simulink model "nonlinear_MPC"  (R2026a)
settings: Solver=ode23s  StopTime=1369
undefined symbols (not defined in the file): acp, bcp, c, ccp, dcp, f, ka, kc, Pamb, R, Ra, T, va, vc
libraries: autolibrcnetworksystem x1, mpclib x1
settings Model: Creator=siddh  LastModifiedBy=siddh

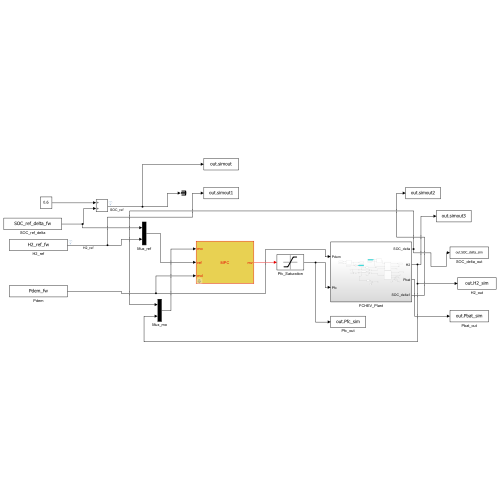
[thumbnail: Simulink's stored preview of the top-level diagram]
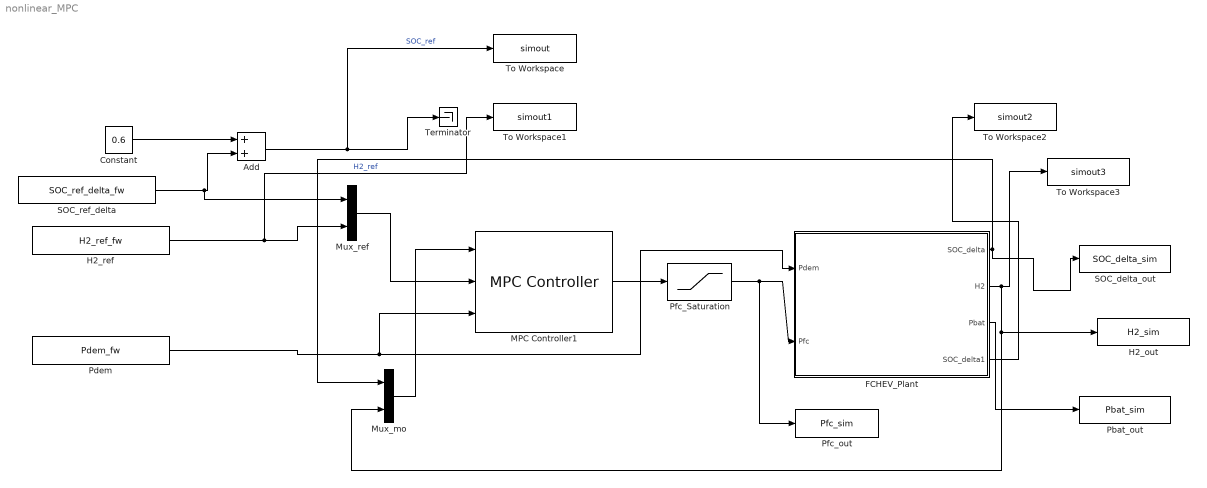
== system nonlinear_MPC ==
  Add : Sum
  Constant : Constant  Value=0.6
  FCHEV_Plant : Subsystem
  H2_out : ToWorkspace  VariableName=H2_sim  SaveFormat=Timeseries  SampleTime=-1
  H2_ref : FromWorkspace  VariableName=H2_ref_fw  SampleTime=-1  OutputAfterFinalValue=Holding final value
  MPC Controller1 : mpclib/MPC Controller  SCDEnableBlockLinearizationSpecification=on  mpcobj=mpcobj  is_multiple=0  enable_value=0  return_u0=off  updateMPCinCallerWorkspace=on  md_inport=on  mv_inport=off  uref_inport=off  return_cost=off  return_mvseq=off  return_qpstatus=off  return_xseq=off  return_state=off  return_ovseq=off  state_inport=off  umin_inport=off  umax_inport=off  ymin_inport=off  ymax_inport=off  cc_inport=off  ywt_inport=off  uwt_inport=off  duwt_inport=off  rhoeps_inport=off  pm_inport=off  MaximumP=10  HorizonChoice=FixedHorizon  n_ts=1  n_p=30  n_mv=1  n_md=1  n_ud=0  n_mo=2  n_uo=0  BlockDataType=double  SampleTimeInherited=off  switch_inport=off
  Mux_mo : Mux  Inputs=2
  Mux_ref : Mux  Inputs=2
  Pbat_out : ToWorkspace  VariableName=Pbat_sim  SaveFormat=Timeseries  SampleTime=-1
  Pdem : FromWorkspace  VariableName=Pdem_fw  SampleTime=-1  OutputAfterFinalValue=Holding final value
  Pfc_Saturation : Saturate  UpperLimit=106000  LowerLimit=0
  Pfc_out : ToWorkspace  VariableName=Pfc_sim  SaveFormat=Timeseries  SampleTime=-1
  SOC_delta_out : ToWorkspace  VariableName=SOC_delta_sim  SaveFormat=Timeseries  SampleTime=-1
  SOC_ref_delta : FromWorkspace  VariableName=SOC_ref_delta_fw  SampleTime=-1  OutputAfterFinalValue=Holding final value
  Terminator : Terminator
  To Workspace : ToWorkspace  VariableName=simout  SaveFormat=Timeseries  SampleTime=-1
  To Workspace1 : ToWorkspace  VariableName=simout1  SaveFormat=Timeseries  SampleTime=-1
  To Workspace2 : ToWorkspace  VariableName=simout2  SaveFormat=Timeseries  SampleTime=-1
  To Workspace3 : ToWorkspace  VariableName=simout3  SaveFormat=Timeseries  SampleTime=-1
  wires:
  H2_ref/1 -> To Workspace1/1, Mux_ref/2  "H2_ref"
  Mux_ref/1 -> MPC Controller1/2
  Pdem/1 -> MPC Controller1/3, FCHEV_Plant/1(Pdem)
  MPC Controller1/1 -> Pfc_Saturation/1
  Pfc_Saturation/1 -> FCHEV_Plant/2(Pfc), Pfc_out/1
  FCHEV_Plant/1(SOC_delta) -> SOC_delta_out/1, Mux_mo/1
  FCHEV_Plant/2(H2) -> To Workspace3/1, Mux_mo/2, H2_out/1
  Mux_mo/1 -> MPC Controller1/1
  FCHEV_Plant/3(Pbat) -> Pbat_out/1
  SOC_ref_delta/1 -> Mux_ref/1, Add/2
  Constant/1 -> Add/1
  Add/1 -> To Workspace/1, Terminator/1  "SOC_ref"
  FCHEV_Plant/4(SOC_delta1) -> To Workspace2/1

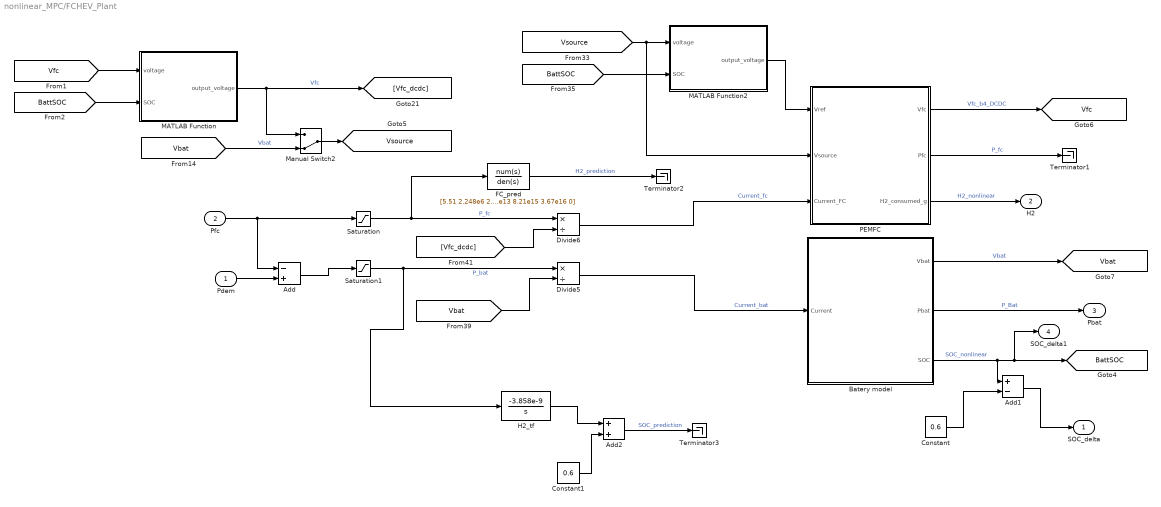
== system nonlinear_MPC/FCHEV_Plant ==
  Pdem : Inport
  Pfc : Inport  Port=2
  Add : Sum  Inputs=-+
  Add1 : Sum  Inputs=+-
  Add2 : Sum
  Batery model : Subsystem
  Constant : Constant  Value=0.6
  Constant1 : Constant  Value=0.6
  Divide5 : Product  Inputs=*/
  Divide6 : Product  Inputs=*/
  FC_pred : TransferFcn  Numerator=[5.51 2.248e6 2.488e9 6.473e11]  Denominator=[1044 1.239e10 2.034e13 8.21e15 3.67e16 0]
  H2_tf : TransferFcn  Numerator=[0 -3.858e-9]  Denominator=[1 0]
  MATLAB Function : MATLAB Function  TreatAsAtomicUnit=on
  MATLAB Function2 : MATLAB Function  TreatAsAtomicUnit=on
  Manual Switch2 : ManualSwitch  CurrentSetting=0
  PEMFC : Subsystem
  Saturation : Saturate  UpperLimit=106000  LowerLimit=0
  Saturation1 : Saturate  UpperLimit=78000  LowerLimit=-78000
  Terminator1 : Terminator
  Terminator2 : Terminator
  Terminator3 : Terminator
  SOC_delta : Outport
  H2 : Outport  Port=2
  Pbat : Outport  Port=3
  SOC_delta1 : Outport  Port=4
  tag scope: BattSOC=global, Vbat=global, Vfc=global, Vsource=global
  wires:
  Pdem/1 -> Add/2
  Pfc/1 -> Saturation/1, Add/1
  MATLAB Function2/1(output_voltage) -> PEMFC/1(Vref)
  [Vbat] -> Divide5/2
  [Vfc] -> MATLAB Function/1(voltage)
  [Vfc_dcdc] -> Divide6/2
  Divide6/1 -> PEMFC/3(Current_FC)  "Current_fc"
  Batery model/3(SOC) -> SOC_delta1/1, [BattSOC], Add1/1  "SOC_nonlinear"
  [BattSOC] -> MATLAB Function/2(SOC)
  [BattSOC] -> MATLAB Function2/2(SOC)
  PEMFC/2(Pfc) -> Terminator1/1  "P_fc"
  [Vsource] -> PEMFC/2(Vsource), MATLAB Function2/1(voltage)
  Saturation/1 -> FC_pred/1, Divide6/1  "P_fc"
  Divide5/1 -> Batery model/1(Current)  "Current_bat"
  Saturation1/1 -> H2_tf/1, Divide5/1  "P_bat"
  Manual Switch2/1 -> [Vsource]
  PEMFC/3(H2_consumed_g) -> H2/1  "H2_nonlinear"
  Batery model/2(Pbat) -> Pbat/1  "P_Bat"
  MATLAB Function/1(output_voltage) -> Manual Switch2/1, [Vfc_dcdc]  "Vfc"
  [Vbat] -> Manual Switch2/2  "Vbat"
  Add/1 -> Saturation1/1
  Constant/1 -> Add1/2
  Add1/1 -> SOC_delta/1
  PEMFC/1(Vfc) -> [Vfc]  "Vfc_b4_DCDC"
  Batery model/1(Vbat) -> [Vbat]  "Vbat"
  FC_pred/1 -> Terminator2/1  "H2_prediction"
  Constant1/1 -> Add2/2
  Add2/1 -> Terminator3/1  "SOC_prediction"
  H2_tf/1 -> Add2/1

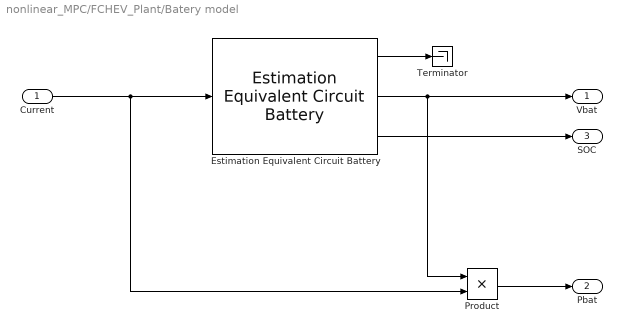
== system nonlinear_MPC/FCHEV_Plant/Batery model ==
  Current : Inport
  Estimation Equivalent Circuit Battery : autolibrcnetworksystem/Estimation Equivalent Circuit Battery  NumRC=2  Em=[650.3 670.3 690.3 720.3 760.3 780.3]  R0=[0.01 0.01 0.01 0.01 0.01 0.01]  SOC_BP=[0 .2 .4 .6 .8 1]  BattCap=100  BattCapInit=100*0.6  InitialCapVoltage=[0 0]  R1=[0.005 0.005 0.005 0.005 0.005 0.005]  C1=[10000 10000 10000 10000 10000 10000]  R2=[0.005 0.005 0.005 0.005 0.005 0.005]  C2=[10000 10000 10000 10000 10000 10000]  R3=[0.005 0.005 0.005 0.005 0.005 0.005]  C3=[10000 10000 10000 10000 10000 10000]  R4=[0.005 0.005 0.005 0.005 0.005 0.005]  C4=[10000 10000 10000 10000 10000 10000]  R5=[0.005 0.005 0.005 0.005 0.005 0.005]  C5=[10000 10000 10000 10000 10000 10000]  Vu=Inf  Vl=-Inf
  Product : Product
  Terminator : Terminator
  Vbat : Outport
  Pbat : Outport  Port=2
  SOC : Outport  Port=3
  wires:
  Current/1 -> Estimation Equivalent Circuit Battery/1, Product/2
  Estimation Equivalent Circuit Battery/1 -> Terminator/1
  Estimation Equivalent Circuit Battery/2 -> Product/1, Vbat/1
  Estimation Equivalent Circuit Battery/3 -> SOC/1
  Product/1 -> Pbat/1

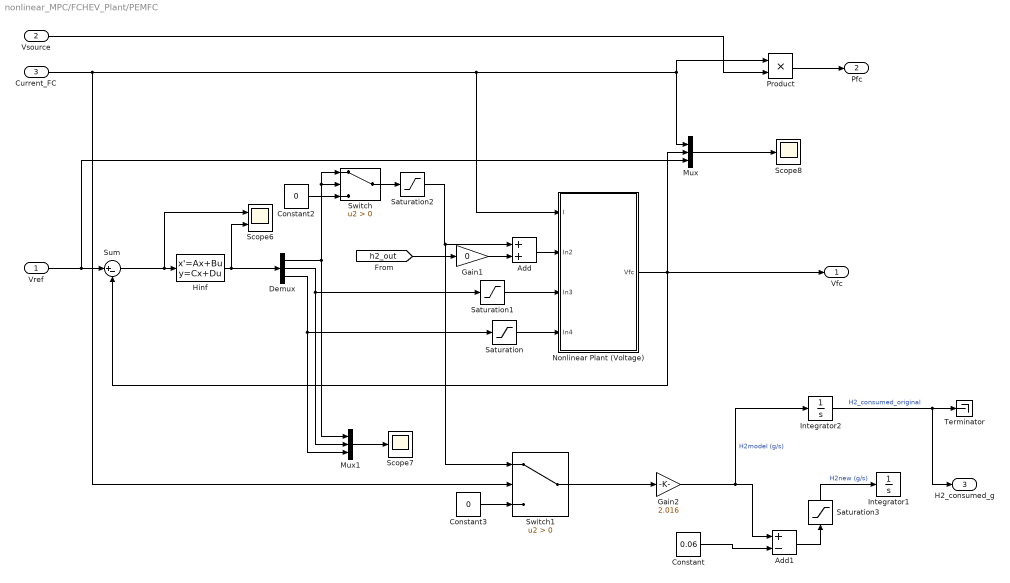
== system nonlinear_MPC/FCHEV_Plant/PEMFC ==
  Vref : Inport
  Vsource : Inport  Port=2
  Current_FC : Inport  Port=3
  Add : Sum
  Add1 : Sum  Inputs=+-
  Constant : Constant  Value=0.06
  Constant2 : Constant  Value=0
  Constant3 : Constant  Value=0
  Demux : Demux  Outputs=3
  Gain1 : Gain  Gain=0
  Gain2 : Gain  Gain=2.016
  Hinf : StateSpace  A=acp  B=bcp  C=ccp  D=dcp  InitialCondition=0
  Integrator1 : Integrator
  Integrator2 : Integrator
  Mux : Mux  Inputs=3
  Mux1 : Mux  Inputs=3
  Nonlinear Plant (Voltage) : Subsystem
  Product : Product
  Saturation{,1..3} (4 alike) : Saturate  UpperLimit=inf  LowerLimit=0
  Scope6 : Scope  NumInputPorts=2
      settings: ActiveDisplayYMinimum=-1.5688075273741493  ActiveDisplayYMaximum=17.817151059973682  DataLoggingVariableName=ScopeData7
  Scope7 : Scope
      settings: ActiveDisplayYMinimum=-0.32178  ActiveDisplayYMaximum=0.56584  DataLoggingVariableName=ScopeData8
  Scope8 : Scope
      settings: ActiveDisplayYMinimum=-55.00153  ActiveDisplayYMaximum=495.01374  DataLoggingVariableName=ScopeData9
  Sum : Sum  Inputs=|+-
  Switch : Switch  Criteria=u2 > Threshold  SaturateOnIntegerOverflow=off  InputSameDT=off
  Switch1 : Switch  Criteria=u2 > Threshold  SaturateOnIntegerOverflow=off  InputSameDT=off
  Terminator : Terminator
  Vfc : Outport
  Pfc : Outport  Port=2
  H2_consumed_g : Outport  Port=3
  wires:
  Mux1/1 -> Scope7/1
  Vref/1 -> Sum/1, Mux/3
  Saturation/1 -> Nonlinear Plant (Voltage)/4(In4)
  Sum/1 -> Scope6/1, Hinf/1
  Mux/1 -> Scope8/1
  Hinf/1 -> Demux/1, Scope6/2
  Demux/3 -> Saturation/1, Mux1/3
  Demux/1 -> Mux1/1, Switch/2, Switch/1
  Nonlinear Plant (Voltage)/1(Vfc) -> Mux/2, Sum/2, Vfc/1
  Saturation1/1 -> Nonlinear Plant (Voltage)/3(In3)
  Demux/2 -> Saturation1/1, Mux1/2
  Saturation2/1 -> Switch1/1, Add/1
  [h2_out] -> Gain1/1
  Gain1/1 -> Add/2
  Add/1 -> Nonlinear Plant (Voltage)/2(In2)
  Constant2/1 -> Switch/3
  Switch/1 -> Saturation2/1
  Product/1 -> Pfc/1
  Vsource/1 -> Product/2
  Switch1/1 -> Gain2/1
  Constant3/1 -> Switch1/3
  Current_FC/1 -> Switch1/2, Nonlinear Plant (Voltage)/1(I), Mux/1, Product/1
  Constant/1 -> Add1/2
  Gain2/1 -> Integrator2/1, Add1/1  "H2model (g/s)"
  Add1/1 -> Saturation3/1
  Saturation3/1 -> Integrator1/1  "H2new (g/s)"
  Integrator2/1 -> H2_consumed_g/1, Terminator/1  "H2_consumed_original"

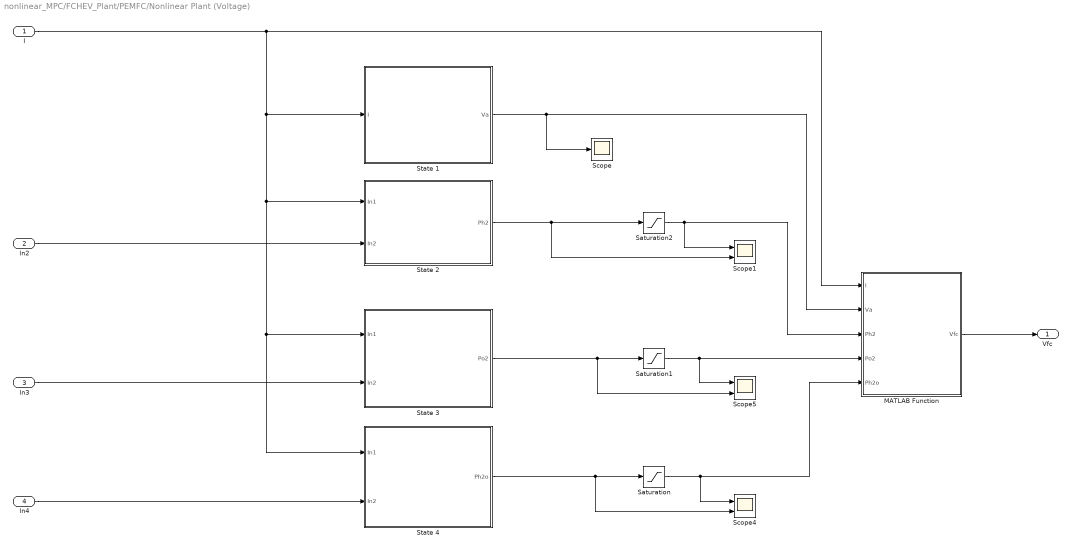
== system nonlinear_MPC/FCHEV_Plant/PEMFC/Nonlinear Plant (Voltage) ==
  I : Inport
  In2 : Inport  Port=2
  In3 : Inport  Port=3
  In4 : Inport  Port=4
  MATLAB Function : MATLAB Function  TreatAsAtomicUnit=on
  Saturation : Saturate  UpperLimit=inf  LowerLimit=1e-9
  Saturation1 : Saturate  UpperLimit=inf  LowerLimit=1e-9
  Saturation2 : Saturate  UpperLimit=inf  LowerLimit=1e-9
  Scope : Scope
      settings: ActiveDisplayYMinimum=-0.0125  ActiveDisplayYMaximum=0.1125
  Scope1 : Scope  NumInputPorts=2
      settings: ActiveDisplayYMinimum=-37.63702  ActiveDisplayYMaximum=338.7332  DataLoggingVariableName=ScopeData5
  Scope4 : Scope  NumInputPorts=2
      settings: ActiveDisplayYMinimum=-2888.51754  ActiveDisplayYMaximum=25996.65787  DataLoggingVariableName=ScopeData2
  Scope5 : Scope  NumInputPorts=2
      settings: ActiveDisplayYMinimum=-0.11528  ActiveDisplayYMaximum=1.03755  DataLoggingVariableName=ScopeData3
  State 1 : Subsystem
  State 2 : Subsystem
  State 3 : Subsystem
  State 4 : Subsystem
  Vfc : Outport
  wires:
  In3/1 -> State 3/2(In2)
  State 1/1(Va) -> Scope/1, MATLAB Function/2(Va)
  I/1 -> MATLAB Function/1(I), State 3/1(In1), State 4/1(In1), State 2/1(In1), State 1/1(I)
  In4/1 -> State 4/2(In2)
  MATLAB Function/1(Vfc) -> Vfc/1
  In2/1 -> State 2/2(In2)
  State 4/1(Ph2o) -> Scope4/2, Saturation/1
  State 3/1(Po2) -> Scope5/2, Saturation1/1
  Saturation/1 -> MATLAB Function/5(Ph2o), Scope4/1
  Saturation1/1 -> MATLAB Function/4(Po2), Scope5/1
  Saturation2/1 -> Scope1/1, MATLAB Function/3(Ph2)
  State 2/1(Ph2) -> Saturation2/1, Scope1/2

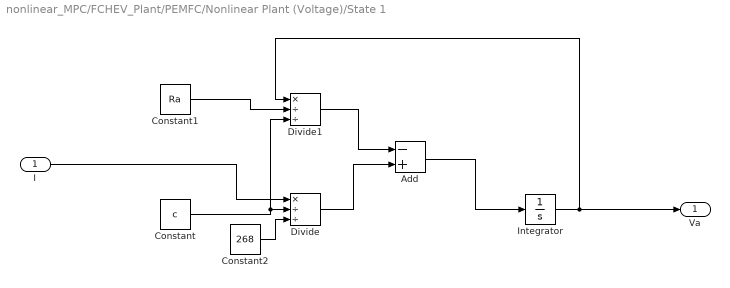
== system nonlinear_MPC/FCHEV_Plant/PEMFC/Nonlinear Plant (Voltage)/State 1 ==
  I : Inport
  Add : Sum  Inputs=-+
  Constant : Constant  Value=c
  Constant1 : Constant  Value=Ra
  Constant2 : Constant  Value=268
  Divide : Product  Inputs=*//
  Divide1 : Product  Inputs=*//
  Integrator : Integrator
  Va : Outport
  wires:
  Add/1 -> Integrator/1
  Integrator/1 -> Va/1, Divide1/1
  Constant1/1 -> Divide1/2
  Constant/1 -> Divide1/3, Divide/2
  Divide1/1 -> Add/1
  I/1 -> Divide/1
  Divide/1 -> Add/2
  Constant2/1 -> Divide/3

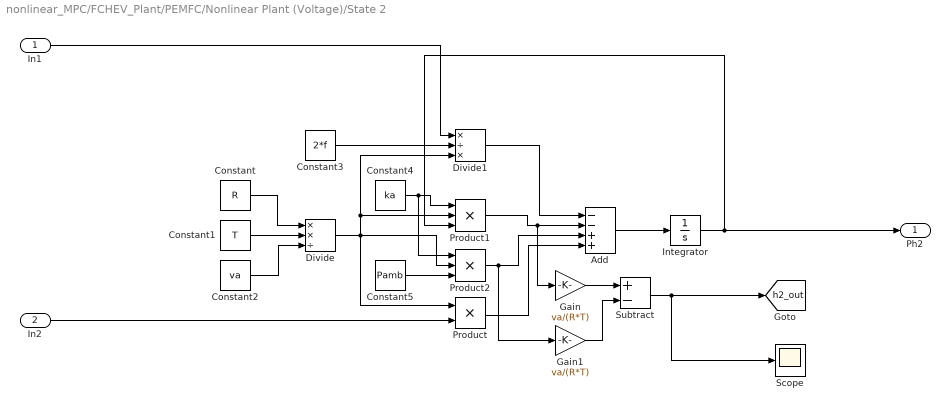
== system nonlinear_MPC/FCHEV_Plant/PEMFC/Nonlinear Plant (Voltage)/State 2 ==
  In1 : Inport
  In2 : Inport  Port=2
  Add : Sum  Inputs=--++
  Constant : Constant  Value=R
  Constant1 : Constant  Value=T
  Constant2 : Constant  Value=va
  Constant3 : Constant  Value=2*f
  Constant4 : Constant  Value=ka
  Constant5 : Constant  Value=Pamb
  Divide : Product  Inputs=**/
  Divide1 : Product  Inputs=*/*
  Gain : Gain  Gain=va/(R*T)
  Gain1 : Gain  Gain=va/(R*T)
  Integrator : Integrator
  Product : Product
  Product1 : Product  Inputs=3
  Product2 : Product  Inputs=3
  Scope : Scope
      settings: ActiveDisplayYMinimum=-0.15455  ActiveDisplayYMaximum=1.35093  DataLoggingVariableName=ScopeData3
  Subtract : Sum  Inputs=+-
  Ph2 : Outport
  tag scope: h2_out=global
  wires:
  Divide/1 -> Product1/2, Divide1/3, Product2/2, Product/1
  Constant4/1 -> Product2/1, Product1/1
  Product1/1 -> Gain/1, Add/2
  Integrator/1 -> Ph2/1, Product1/3
  Product/1 -> Add/4
  Constant1/1 -> Divide/2
  In2/1 -> Product/2
  Constant2/1 -> Divide/3
  Divide1/1 -> Add/1
  Product2/1 -> Gain1/1, Add/3
  Constant3/1 -> Divide1/2
  Constant/1 -> Divide/1
  Add/1 -> Integrator/1
  Constant5/1 -> Product2/3
  In1/1 -> Divide1/1
  Subtract/1 -> Scope/1, [h2_out]
  Gain/1 -> Subtract/1
  Gain1/1 -> Subtract/2

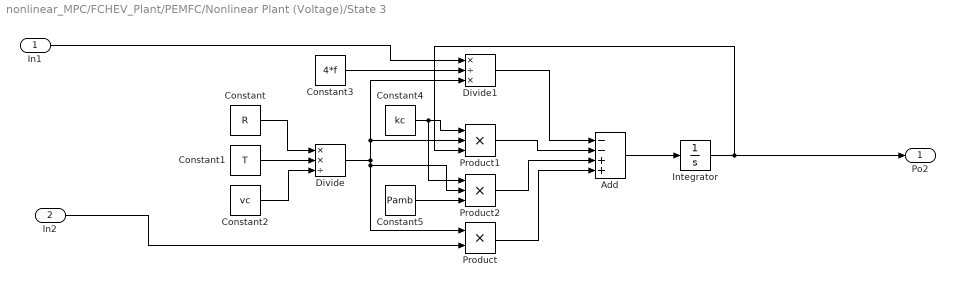
== system nonlinear_MPC/FCHEV_Plant/PEMFC/Nonlinear Plant (Voltage)/State 3 ==
  In1 : Inport
  In2 : Inport  Port=2
  Add : Sum  Inputs=--++
  Constant : Constant  Value=R
  Constant1 : Constant  Value=T
  Constant2 : Constant  Value=vc
  Constant3 : Constant  Value=4*f
  Constant4 : Constant  Value=kc
  Constant5 : Constant  Value=Pamb
  Divide : Product  Inputs=**/
  Divide1 : Product  Inputs=*/*
  Integrator : Integrator
  Product : Product
  Product1 : Product  Inputs=3
  Product2 : Product  Inputs=3
  Po2 : Outport
  wires:
  Divide1/1 -> Add/1
  Constant5/1 -> Product2/3
  Integrator/1 -> Po2/1, Product1/3
  Constant4/1 -> Product2/1, Product1/1
  Divide/1 -> Product2/2, Product/1, Product1/2, Divide1/3
  Constant/1 -> Divide/1
  In2/1 -> Product/2
  Add/1 -> Integrator/1
  Constant2/1 -> Divide/3
  Product1/1 -> Add/2
  Constant3/1 -> Divide1/2
  Product2/1 -> Add/3
  Constant1/1 -> Divide/2
  Product/1 -> Add/4
  In1/1 -> Divide1/1

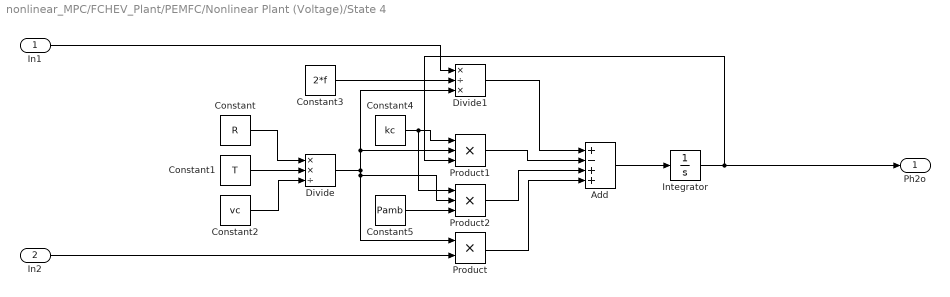
== system nonlinear_MPC/FCHEV_Plant/PEMFC/Nonlinear Plant (Voltage)/State 4 ==
  In1 : Inport
  In2 : Inport  Port=2
  Add : Sum  Inputs=+-++
  Constant : Constant  Value=R
  Constant1 : Constant  Value=T
  Constant2 : Constant  Value=vc
  Constant3 : Constant  Value=2*f
  Constant4 : Constant  Value=kc
  Constant5 : Constant  Value=Pamb
  Divide : Product  Inputs=**/
  Divide1 : Product  Inputs=*/*
  Integrator : Integrator
  Product : Product
  Product1 : Product  Inputs=3
  Product2 : Product  Inputs=3
  Ph2o : Outport
  wires:
  Constant5/1 -> Product2/3
  Divide1/1 -> Add/1
  Divide/1 -> Product2/2, Product/1, Product1/2, Divide1/3
  Integrator/1 -> Ph2o/1, Product1/3
  In2/1 -> Product/2
  Product1/1 -> Add/2
  Add/1 -> Integrator/1
  Constant4/1 -> Product2/1, Product1/1
  Constant/1 -> Divide/1
  Constant3/1 -> Divide1/2
  Product/1 -> Add/4
  Constant2/1 -> Divide/3
  Product2/1 -> Add/3
  Constant1/1 -> Divide/2
  In1/1 -> Divide1/1

== matlab function nonlinear_MPC/FCHEV_Plant/PEMFC/Nonlinear Plant (Voltage)/MATLAB Function ==
  data: I input; Vfc output; Va input; Ph2 input; Po2 input; Ph2o input
function Vfc = fcn(I,Va,Ph2,Po2,Ph2o)
Vfc = 436*(1.105 + (8.314*333/(2*96485))*log((Ph2)*(Po2)^(0.5)/(Ph2o))-Va-(0.14*(I/268+1)));
end

== matlab function nonlinear_MPC/FCHEV_Plant/MATLAB Function2 ==
  data: voltage input; output_voltage output; SOC input

function output_voltage = Inv_DCDCGain(voltage, SOC)
%#codegen
    % Define SOC values and corresponding gains
    SOC_values = [0, 0.2, 0.4, 0.6, 0.8, 1];
    gains = [1.4780, 1.5234, 1.5689, 1.6370, 1.7280, 1.7734];
    
    % Interpolate gain based on SOC input
    gain = interp1(SOC_values, gains, SOC(1), 'linear', 'extrap');
    
    % Multiply the voltage by the interpolated gain
    output_voltage = voltage * 1/gain;
end

== matlab function nonlinear_MPC/FCHEV_Plant/MATLAB Function ==
  data: voltage input; SOC input; output_voltage output
function output_voltage = DCDCGain(voltage, SOC)
%#codegen
    % Define SOC values and corresponding gains
    SOC_values = [0, 0.2, 0.4, 0.6, 0.8, 1];
    %gains = [1.47, 1.52, 1.56, 1.63, 1.72, 1.77];
    gains = [1.4780    1.5234    1.5689    1.6370    1.7280    1.7734];
    % Interpolate gain based on SOC input
    gain = interp1(SOC_values, gains, SOC(1), 'linear', 'extrap');
    
    % Multiply the voltage by the interpolated gain
    output_voltage = voltage * gain;
end
